simulink model "ace_cl_arduino"  (R2026a)
settings: Solver=FixedStepDiscrete  StopTime=C.cl_T  FixedStep=0.02  EnableMultiTasking=on
PreLoadFcn:
  | ace_params;
InitFcn:
  | ace_params;
values from neighbouring files (symbols this model uses):
  C = struct()    [ace_params.m]    (also in build_ace_sysid_pipeline.m = evalin('base', 'C'))
libraries: arduinolib x3, arduinosensorlib x1, slpidlib x1
settings Model: SimulationMode=external  SILPILModeSetting=veronly  ExtModeTrigDuration=2  Creator=00782620  LastModifiedBy=00782620
settings HardwareCC: ProdBitPerInt=16.0  ProdBitPerPointer=16.0  ProdBitPerSizeT=16.0  ProdBitPerPtrDiffT=16.0  ProdWordSize=8.0  ProdHWDeviceType=Atmel->AVR
settings RTWCC: SystemTargetFile=ert.tlc  HardwareBoard=Arduino Uno  TLCOptions=-aInlineSetEventsForThisBaseRateFcn=TLC_FALSE -aSuppressMultiTaskScheduler=TLC_FALSE -aRateBasedStepFcn=1  Toolchain=Arduino AVR  BuildConfiguration=Faster Runs  Description=Embedded Coder
settings ERTTargetCC: ExtModeTransport=3.0  ExtModeAutomaticAllocSize=off  ExtModeStaticAllocSize=250.0  SupportContinuousTime=on  SupportVariableSizeSignals=on

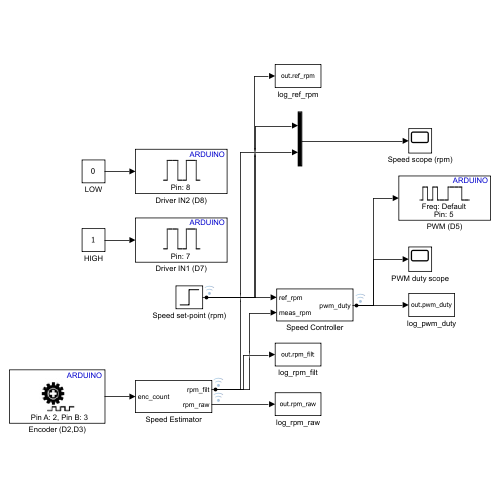
[thumbnail: Simulink's stored preview of the top-level diagram]
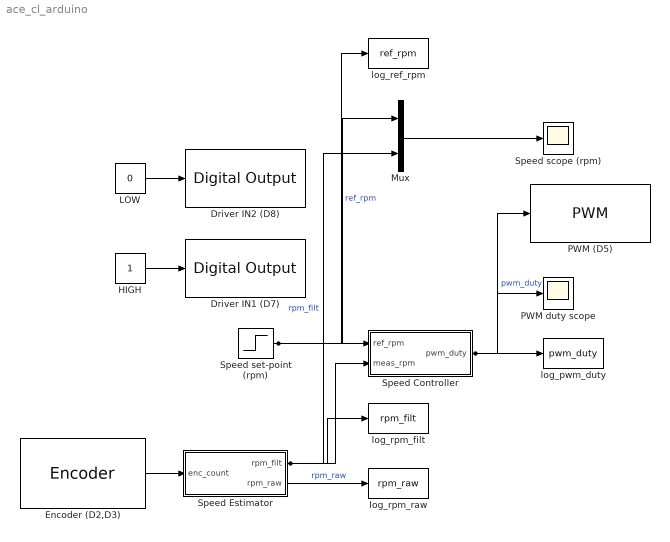
== system ace_cl_arduino ==
  Driver IN1 (D7) : arduinolib/Digital Output  pinNumber=7  Direction=output  blockPlatform=arduino
  Driver IN2 (D8) : arduinolib/Digital Output  pinNumber=8  Direction=output  blockPlatform=arduino
  Encoder (D2,D3) : arduinosensorlib/Encoder  InputA=2  InputB=3  Mode=No reset  SampleTime=0.02
  HIGH : Constant  SampleTime=C.Ts
  LOW : Constant  Value=0  SampleTime=C.Ts
  Mux : Mux  Inputs=2
  PWM (D5) : arduinolib/PWM  pinNumber=5  frequencyType=Default  desiredFrequency=490.2  achievableFrequency=490.2
  PWM duty scope : Scope
  Speed Controller : Subsystem
  Speed Estimator : Subsystem
  Speed scope (rpm) : Scope
  Speed set-point (rpm) : Step  Time=C.t_step_hw  FinalValue=C.ref_rpm  SampleTime=C.Ts
  log_pwm_duty : ToWorkspace  VariableName=pwm_duty  SaveFormat=Timeseries  SampleTime=-1
  log_ref_rpm : ToWorkspace  VariableName=ref_rpm  SaveFormat=Timeseries  SampleTime=-1
  log_rpm_filt : ToWorkspace  VariableName=rpm_filt  SaveFormat=Timeseries  SampleTime=-1
  log_rpm_raw : ToWorkspace  VariableName=rpm_raw  SaveFormat=Timeseries  SampleTime=-1
  wires:
  Speed Estimator/1(rpm_filt) -> Speed Controller/2(meas_rpm), log_rpm_filt/1, Mux/2  "rpm_filt"
  LOW/1 -> Driver IN2 (D8)/1
  Speed Controller/1(pwm_duty) -> log_pwm_duty/1, PWM (D5)/1, PWM duty scope/1  "pwm_duty"
  Mux/1 -> Speed scope (rpm)/1
  HIGH/1 -> Driver IN1 (D7)/1
  Encoder (D2,D3)/1 -> Speed Estimator/1(enc_count)
  Speed set-point (rpm)/1 -> Speed Controller/1(ref_rpm), log_ref_rpm/1, Mux/1  "ref_rpm"
  Speed Estimator/2(rpm_raw) -> log_rpm_raw/1  "rpm_raw"

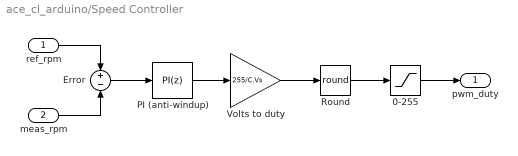
== system ace_cl_arduino/Speed Controller ==
  ref_rpm : Inport
  meas_rpm : Inport  Port=2
  0-255 : Saturate  UpperLimit=255  LowerLimit=0
  Error : Sum  Inputs=+-
  PI (anti-windup) : slpidlib/PID Controller  Controller=PI  Form=Parallel  TimeDomain=Discrete-time  UseExternalTs=off  SampleTime=C.Ts  IntegratorMethod=Forward Euler  FilterMethod=Forward Euler  ControllerParametersSource=internal  P=C.Kp  I=C.Ki  UseKiTs=off  D=0  UseExternalDerivativeSource=off  N=100  UseFilter=on  TunerSelectOption=Transfer Function Based (PID Tuner App)  InitialConditionSource=internal  InitialConditionForIntegrator=0  InitialConditionForFilter=0  DifferentiatorICPrevScaledInput=0  ExternalReset=none  TrackingMode=off  Kt=1  LimitOutput=on  SatLimitsSource=internal  UpperSaturationLimit=C.Vs  LowerSaturationLimit=0  LinearizeAsGain=off  AntiWindupMode=clamping  Kb=1  LimitIntegrator=off  UpperIntegratorSaturationLimit=inf  LowerIntegratorSaturationLimit=-inf  POutMin=[]  POutMax=[]  IOutMin=[]  IOutMax=[]  DOutMin=[]  DOutMax=[]  NOutMin=[]  NOutMax=[]  SumOutMin=[]  SumOutMax=[]  SaturationOutMin=[]  SaturationOutMax=[]  PParamMin=[]  PParamMax=[]  IParamMin=[]  IParamMax=[]  DParamMin=[]  DParamMax=[]  NParamMin=[]  NParamMax=[]  KbParamMin=[]  KbParamMax=[]  KtParamMin=[]  KtParamMax=[]  KbOutMin=[]  KbOutMax=[]  KtOutMin=[]  KtOutMax=[]  IntegratorOutMin=[]  IntegratorOutMax=[]  FilterOutMin=[]  FilterOutMax=[]  SumI1OutMin=[]  SumI1OutMax=[]  SumI2OutMin=[]  SumI2OutMax=[]  SumI3OutMin=[]  SumI3OutMax=[]  SumI4OutMin=[]  SumI4OutMax=[]  SumDOutMin=[]  SumDOutMax=[]  DifferentiatorOutMin=[]  DifferentiatorOutMax=[]  FilterDiffOutCoefMin=[]  FilterDiffOutCoefMax=[]  ReciprocalOutMin=[]  ReciprocalOutMax=[]  SumDenOutMin=[]  SumDenOutMax=[]  SumNumOutMin=[]  SumNumOutMax=[]  DivideOutMin=[]  DivideOutMax=[]  UdiffTsProdOutMin=[]  UdiffTsProdOutMax=[]  NTsProdOutMin=[]  NTsProdOutMax=[]  UintegralTsProdOutMin=[]  UintegralTsProdOutMax=[]  UngainTsProdOutMin=[]  UngainTsProdOutMax=[]  ClampingZeroOutDataTypeStr=Inherit: Inherit via back propagation  ClampingZeroOutMin=[]  ClampingZeroOutMax=[]  FilterDenConstantOutDataTypeStr=Inherit: Inherit via back propagation  FilterDenConstantOutMin=[]  FilterDenConstantOutMax=[]  PCopyOutDataTypeStr=Inherit: Inherit via back propagation  PCopyOutMin=[]  PCopyOutMax=[]  NCopyOutDataTypeStr=Inherit: Inherit via back propagation  NCopyOutMin=[]  NCopyOutMax=[]  IntegratorContinuousStateAttributes=''  IntegratorStateMustResolveToSignalObject=off  IntegratorRTWStateStorageClass=Auto  FilterContinuousStateAttributes=''  FilterStateMustResolveToSignalObject=off  FilterRTWStateStorageClass=Auto  ParallelPVariant=InternalParameters  IdealPVariant=Disabled  IVariant=InternalParameters  DVariant=Disabled  IntegratorVariant=Discrete  SatVariant=Enabled  AWVariant=DiscClampingParallel  PCopyVariant=Disabled  TRVariant=Disabled  FdbkBlocksVariant=Forward  IdealPFdbkVariant=Disabled  SatFdbkVariant=Disabled  DerivativeFilterVariant=Disabled  NVariant=Disabled  NCopyVariant=Disabled_SignalSpec  FilterICVariant=Disabled  IntegratorICVariant=InternalICs  ExternalResetVariant=Disabled  TRSumVariant=Passthrough  SumFdbkVariant=Disabled  SumVariant=Sum_PI  TsampFilterVariant=InternalTs  TsampNgainVariant=Passthrough  TsampIntegralVariant=Disabled_SignalSpec  ExternalSaturationOutDataTypeStr=Inherit: Same as second input  DerivativeSourceVariant=Disabled  PreIntVariant=InternalPreInt
      settings: LibrarySourceBlock=simulink/Discrete/Discrete PID Controller
  Round : Rounding  Operator=round
  Volts to duty : Gain  Gain=255/C.Vs
  pwm_duty : Outport
  wires:
  Round/1 -> 0-255/1
  ref_rpm/1 -> Error/1
  Error/1 -> PI (anti-windup)/1
  meas_rpm/1 -> Error/2
  PI (anti-windup)/1 -> Volts to duty/1
  Volts to duty/1 -> Round/1
  0-255/1 -> pwm_duty/1

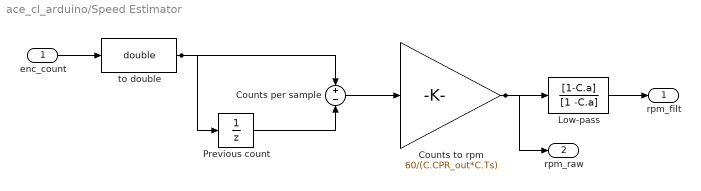
== system ace_cl_arduino/Speed Estimator ==
  enc_count : Inport
  Counts per sample : Sum  Inputs=+-
  Counts to rpm : Gain  Gain=60/(C.CPR_out*C.Ts)
  Low-pass : DiscreteTransferFcn  Numerator=[1-C.a]  Denominator=[1 -C.a]  SampleTime=C.Ts
  Previous count : UnitDelay  SampleTime=C.Ts
  to double : DataTypeConversion  OutDataTypeStr=double  SaturateOnIntegerOverflow=off  RndMeth=Floor
  rpm_filt : Outport
  rpm_raw : Outport  Port=2
  wires:
  Counts to rpm/1 -> rpm_raw/1, Low-pass/1
  Counts per sample/1 -> Counts to rpm/1
  Previous count/1 -> Counts per sample/2
  enc_count/1 -> to double/1
  to double/1 -> Counts per sample/1, Previous count/1
  Low-pass/1 -> rpm_filt/1
